simulink model "turbo_controller"  (R2025a)
settings: Solver=FixedStepAuto  StartTime=0.0  StopTime=inf  FixedStep=0.001  RelTol=1e-3
PostLoadFcn:
  | % 自动定位同目录CubeMX文件；不需要外部初始化脚本。
  | codertarget.data.setParameterValue('turbo_controller','STM32CubeMX.ProjectFile',fullfile(fileparts(get_param('turbo_controller','FileName')),'turbo_f407.ioc'));
InitFcn:
  | % 中文说明：按原控制器字段与类型创建三组接口总线；控制参数已内嵌。
  | tc_names=["EValve_Cycle" "EValve_Open" "Eblast_Cycle" "Eblast_Open" "Motor_Cycle" "Motor_Open" "EValve_Enable" "Eblast_Enable" "Motor_Enable" "SWO_Firework" "SWO_BleedAir" "EngineState" "Flag_ECUReset_Clear" "Flag_ECUReset_Save" "Flag_Reset_Enable" "Accelerator" "Nc_dem" "Nc"]; tc_types=["uint16" "uint16" "uint16" "uint16" "uint16" "uint16" "uint8" "uint8" "uint8" "uint8" "uint8" "uint8" "uint8" "uint8" "uint8" "single" "single" "single"];
  | for tc_k=1:numel(tc_names)
  |  tc_e(tc_k)=Simulink.BusElement; tc_e(tc_k).Name=char(tc_names(tc_k)); tc_e(tc_k).DataType=char(tc_types(tc_k));
  | end
  | EngineControl_Out=Simulink.Bus; EngineControl_Out.DataScope='Exported'; EngineControl_Out.Elements=tc_e;
  | clear tc_e tc_names tc_types tc_k
  | tc_names=["savedata1" "savedata2" "savedata3" "savedata4" "savedata5" "savedata6" "savedata7" "savedata8" "savedata9" "savedata10" "savedata11" "savedata12" "savedata13" "savedata14" "savedata15" "savedata16" "savedata17" "savedata18" "savedata19" "savedata20" "savedata21" "savedata22" "savedata23" "savedata24" "savedata25"]; tc_types=["single" "single" "single" "single" "single" "single" "single" "single" "single" "single" "single" "single" "single" "single" "single" "single" "single" "single" "single" "single" "single" "single" "single" "single" "single"];
  | for tc_k=1:numel(tc_names)
  |  tc_e(tc_k)=Simulink.BusElement; tc_e(tc_k).Name=char(tc_names(tc_k)); tc_e(tc_k).DataType=char(tc_types(tc_k));
  | end
  | SaveData_Out=Simulink.Bus; SaveData_Out.DataScope='Exported'; SaveData_Out.Elements=tc_e;
  | clear tc_e tc_names tc_types tc_k
  | tc_names=["senddata1" "senddata2" "senddata3" "senddata4" "senddata5" "senddata6" "senddata7" "senddata8" "senddata9" "senddata10" "senddata11" "senddata12" "senddata13" "senddata14" "senddata15" "senddata16" "senddata17" "senddata18" "senddata19" "senddata20" "senddata21" "senddata22" "senddata23" "senddata24" "senddata25" "senddata26" "senddata27" "senddata28" "senddata29"]; tc_types=["uint8" "uint8" "uint8" "uint8" "uint8" "uint8" "uint8" "uint8" "uint8" "uint8" "uint8" "uint8" "uint8" "uint8" "uint8" "uint8" "uint8" "uint8" "uint8" "uint8" "uint8" "uint8" "uint8" "uint8" "uint8" "uint8" "uint8" "uint8" "uint8"];
  | for tc_k=1:numel(tc_names)
  |  tc_e(tc_k)=Simulink.BusElement; tc_e(tc_k).Name=char(tc_names(tc_k)); tc_e(tc_k).DataType=char(tc_types(tc_k));
  | end
  | SendData_Out=Simulink.Bus; SendData_Out.DataScope='Exported'; SendData_Out.Elements=tc_e;
  | clear tc_e tc_names tc_types tc_k
  | 
  | % 以下为接口中文说明；只设置描述，不改变数值或数据类型。
  | EngineControl_Out.Description='执行控制输出（阀、电机、点火、状态及复位请求）';
  | tc_cn=["EValve_Cycle（主油阀周期计数（每计数2毫秒））" "EValve_Open（主油阀开通计数（每计数2毫秒））" "Eblast_Cycle（副油阀周期计数（每计数2毫秒））" "Eblast_Open（副油阀开通计数（每计数2毫秒））" "Motor_Cycle（起动电机周期计数）" "Motor_Open（起动电机开通计数）" "EValve_Enable（主油阀驱动使能）" "Eblast_Enable（副油阀驱动使能）" "Motor_Enable（起动电机使能）" "SWO_Firework（点火器使能（1开））" "SWO_BleedAir（引气阀使能（1开））" "EngineState（发动机状态）" "Flag_ECUReset_Clear（清除复位恢复状态请求）" "Flag_ECUReset_Save（保存复位恢复数据请求）" "Flag_Reset_Enable（处理器软件复位请求）" "Accelerator（油门／油泵给定控制量）" "Nc_dem（控制目标转速）" "Nc（发动机反馈转速（转每分））"];
  | tc_elements=EngineControl_Out.Elements;
  | for tc_k=1:numel(tc_cn)
  |  tc_elements(tc_k).Description=char(tc_cn(tc_k));
  | end
  | EngineControl_Out.Elements=tc_elements;
  | clear tc_cn tc_elements tc_k
  | SaveData_Out.Description='25项运行记录；字段含义按当前模型数据来源解释';
  | tc_cn=["savedata1（指令回显记录）" "savedata2（入口总温记录（℃））" "savedata3（电源电压记录）" "savedata4（排气温度记录（℃））" "savedata5（标定燃油压力记录）" "savedata6（副油阀占空比记录（％））" "savedata7（主油阀占空比记录（％））" "savedata8（温度修正转速记录）" "savedata9（开关输出及反馈位域）" "savedata10（物理转速记录）" "savedata11（油泵目标给定原始值）" "savedata12（起动电机占空比记录（％））" "savedata13（发动机状态码记录）" "savedata14（故障告警位域记录）" "savedata15（模型记录帧序号）" "savedata16（处理器温度记录（℃））" "savedata17（装订转速记录（沿用旧电源字段名））" "savedata18（导航高度记录）" "savedata19（飞行空速记录）" "savedata20（主阀旧记录位（恒零保留））" "savedata21（第21项保留记录（恒零））" "savedata22（保留记录项22）" "savedata23（保留记录项23）" "savedata24（保留记录项24）" "savedata25（保留记录项25）"];
  | tc_elements=SaveData_Out.Elements;
  | for tc_k=1:numel(tc_cn)
  |  tc_elements(tc_k).Description=char(tc_cn(tc_k));
  | end
  | SaveData_Out.Elements=tc_elements;
  | clear tc_cn tc_elements tc_k
  | SendData_Out.Description='29字段回传及外设命令接口；板端上位机帧只取第3至27字段';
  | tc_cn=["senddata1（回传发送允许标志（不直接上线路））" "senddata2（回传载荷长度25字节）" "senddata3（回传指令回显字节）" "senddata4（总温编码字节（℃＋80））" "senddata5（电源电压编码字节）" "senddata6（排温编码高字节）" "senddata7（排温编码低字节）" "senddata8（燃油压力编码高字节）" "senddata9（燃油压力编码低字节）" "senddata10（副油阀占空比字节（％））" "senddata11（主油阀占空比字节（％））" "senddata12（修正转速编码高字节）" "senddata13（修正转速编码低字节）" "senddata14（驱动及反馈状态位域）" "senddata15（物理转速编码高字节）" "senddata16（物理转速编码低字节）" "senddata17（油泵目标给定高字节（串口二使用））" "senddata18（油泵目标给定低字节（串口二使用））" "senddata19（起动电机占空比命令（串口一使用））" "senddata20（发动机状态码字节）" "senddata21（故障告警位域字节）" "senddata22（帧序号占位（板端另行填写））" "senddata23（处理器温度编码（℃＋50））" "senddata24（控制目标转速编码高字节）" "senddata25（控制目标转速编码低字节）" "senddata26（占位字节（板端改填实测泵速高字节））" "senddata27（占位字节（板端改填实测泵速低字节））" "senddata28（装订转速高字节（本板未发送））" "senddata29（装订转速低字节（本板未发送））"];
  | tc_elements=SendData_Out.Elements;
  | for tc_k=1:numel(tc_cn)
  |  tc_elements(tc_k).Description=char(tc_cn(tc_k));
  | end
  | SendData_Out.Elements=tc_elements;
  | clear tc_cn tc_elements tc_k
  | 
  | 
  | % FRAM模块化事务：接口类型和上电初始状态，随模型保存，无外部初始化文件。
  | clear FM_elements
  | FM_elements(1)=Simulink.BusElement;FM_elements(1).Name='phase';FM_elements(1).DataType='uint8';FM_elements(1).Dimensions=[1 1];FM_elements(1).Description='phase（当前事务阶段）';
  | FM_elements(2)=Simulink.BusElement;FM_elements(2).Name='a';FM_elements(2).DataType='uint8';FM_elements(2).Dimensions=[64 1];FM_elements(2).Description='a（启动时缓存的首区64字节）';
  | FM_elements(3)=Simulink.BusElement;FM_elements(3).Name='active';FM_elements(3).DataType='uint16';FM_elements(3).Dimensions=[1 1];FM_elements(3).Description='active（当前有效记录区地址）';
  | FM_elements(4)=Simulink.BusElement;FM_elements(4).Name='generation';FM_elements(4).DataType='uint32';FM_elements(4).Dimensions=[1 1];FM_elements(4).Description='generation（当前有效记录代号）';
  | FM_elements(5)=Simulink.BusElement;FM_elements(5).Name='record';FM_elements(5).DataType='uint8';FM_elements(5).Dimensions=[64 1];FM_elements(5).Description='record（本次冻结的待写记录）';
  | FM_elements(6)=Simulink.BusElement;FM_elements(6).Name='addr';FM_elements(6).DataType='uint16';FM_elements(6).Dimensions=[1 1];FM_elements(6).Description='addr（本次备用写入地址）';
  | FM_elements(7)=Simulink.BusElement;FM_elements(7).Name='lastSave';FM_elements(7).DataType='single';FM_elements(7).Dimensions=[1 1];FM_elements(7).Description='lastSave（上次开始保存的秒数）';
  | FM_elements(8)=Simulink.BusElement;FM_elements(8).Name='lastState';FM_elements(8).DataType='uint8';FM_elements(8).Dimensions=[1 1];FM_elements(8).Description='lastState（上次保存时的发动机状态）';
  | FM_elements(9)=Simulink.BusElement;FM_elements(9).Name='boot';FM_elements(9).DataType='boolean';FM_elements(9).Dimensions=[1 1];FM_elements(9).Description='boot（启动记录是否允许恢复）';
  | FM_elements(10)=Simulink.BusElement;FM_elements(10).Name='consumed';FM_elements(10).DataType='boolean';FM_elements(10).Dimensions=[1 1];FM_elements(10).Description='consumed（本次启动恢复通知是否已发送）';
  | FM_elements(11)=Simulink.BusElement;FM_elements(11).Name='payload';FM_elements(11).DataType='uint8';FM_elements(11).Dimensions=[20 1];FM_elements(11).Description='payload（当前20字节恢复内容）';
  | ... (+35 lines)
model workspace (MAT data in the model file):
  CRC16_Table_Reference = [0 4129 8258 12387 16516 20645 24774 28903 33032 37161 41290 45419 ... (256 elements, 256x1)]
  PE_Kaer = [0.15402 0.15402 0.12264 0.10076 0.09481 0.07601 0.07111 0.0569 0.05198 0.04926 0.05308 0.04325 ... (13 elements, 1x13)]
  PE_Nr = [21.2982 61.4260372 67.7475458 72.7394382 76.845934 80.6988798 83.8449282 86.6491912 88.9382406 89.178606 91.1938214 93.4068058 ... (13 elements, 1x13)]
  PE_Pump_Translate = 33.5999984741
  PE_RotaSpeed_Translate = 860
  PE_Taer = [0.4939154 0.4939154 0.40780982 0.34066978 0.31622756 0.30405716 0.34300244 0.26785022 0.37393554 0.23914836 0.44563948 0.31044662 ... (13 elements, 1x13)]
  PF_ACCFULLRANGE = 3360
  PF_Flag_ECUReset = 0
  PF_Flag_rx_suc = 1
  PF_Gear_Info = [40000; 45000; 50000; 55000; 57000; 59000; 60000; 61000; 61000; 61000; 61000; 61000]
  PF_K_TiaoJie = 1
  PF_Kpu = 10
  PF_MySet_Rxdata = [0 0 0 0 0 0 0 0 0 0 0 0 ... (50 elements, 50x1)]
  PF_MyUsart1_Rxdata = [0 0 0 0 0 0 0 0 0 0 0 0 ... (50 elements, 50x1)]
  PF_MyUsart2_Rxdata = [0 0 0 0 0 0 0 0 0 0 0 0 ... (50 elements, 50x1)]
  PF_Reset_Information = [0 0 0 0 0 0 0 0 0 0 0 0 ... (20 elements, 20x1)]
  PF_Sensor_X1_T4 = [0 4095]
  PF_Sensor_X2_T4 = [0 1.66666698456]
  PF_Sensor_X3_T4 = [0 504 999 1497 2010 2529 3051 3568 4076 4571 4959]
  PF_Sensor_X_P2 = [0.5 3]
  PF_Sensor_X_Poil = [0.5 3]
  PF_Sensor_X_T1t = [-50 300]
  PF_Sensor_X_Vpower = [0 3]
  PF_Sensor_X_Vpump = [0 3]
  PF_Sensor_Y1_T4 = [0 3]
  PF_Sensor_Y2_T4 = [0 5000]
  PF_Sensor_Y3_T4 = [0 100 200 300 400 500 600 700 800 900 980]
  PF_Sensor_Y_P2 = [0 1000]
  PF_Sensor_Y_Poil = [0 1000]
  PF_Sensor_Y_T1t = [-50 300]
  PF_Sensor_Y_Vpower = [0 33]
  PF_Sensor_Y_Vpump = [0 33]
  PG_CtrlMode_CloseLoop : mpt.Parameter (value not decoded)
  PG_CtrlMode_ManualAcc : mpt.Parameter (value not decoded)
  PG_CtrlMode_Origin : mpt.Parameter (value not decoded)
  PG_CtrlMode_Start : mpt.Parameter (value not decoded)
  PG_CtrlMode_Stop : mpt.Parameter (value not decoded)
  PG_ES_Clp : mpt.Parameter (value not decoded)
  PG_ES_EngStart : mpt.Parameter (value not decoded)
  PG_ES_Manual : mpt.Parameter (value not decoded)
  PG_ES_Origin : mpt.Parameter (value not decoded)
  PG_ES_Stop : mpt.Parameter (value not decoded)
  PG_Instr_BleedAirSet : mpt.Parameter (value not decoded)
  PG_Instr_CloseLoop : mpt.Parameter (value not decoded)
  PG_Instr_ECUReSet : mpt.Parameter (value not decoded)
  PG_Instr_EValveSet : mpt.Parameter (value not decoded)
  PG_Instr_EblastSet : mpt.Parameter (value not decoded)
  PG_Instr_Erase : mpt.Parameter (value not decoded)
  PG_Instr_FireWorkSet : mpt.Parameter (value not decoded)
  PG_Instr_ManualPlus : mpt.Parameter (value not decoded)
  PG_Instr_ManualrReduce : mpt.Parameter (value not decoded)
  PG_Instr_MotorSet : mpt.Parameter (value not decoded)
  PG_Instr_OilSet : mpt.Parameter (value not decoded)
  PG_Instr_SelfCheck : mpt.Parameter (value not decoded)
  PG_Instr_Start : mpt.Parameter (value not decoded)
  PG_Instr_Stop : mpt.Parameter (value not decoded)
  PG_Instr_StopZero : Simulink.Parameter (value not decoded)
  PG_Location_Air : Simulink.Parameter (value not decoded)
  PG_Location_Gnd : Simulink.Parameter (value not decoded)
  PG_ServoCtrlMode_CloseLoop : Simulink.Parameter (value not decoded)
  PG_ServoCtrlMode_CloseLoopMax : Simulink.Parameter (value not decoded)
  PG_ServoCtrlMode_CloseLoopMin : Simulink.Parameter (value not decoded)
  PG_ServoCtrlMode_ManualAcc : Simulink.Parameter (value not decoded)
  PG_ServoCtrlMode_ManualAccMax : Simulink.Parameter (value not decoded)
  PG_ServoCtrlMode_ManualAccMin : Simulink.Parameter (value not decoded)
  PG_SpeedDot_Permit : Simulink.Parameter (value not decoded)
  PL_EngineModel_Actuator = [0 10 100]
  PL_EngineModel_EngineStar_Press_P2 = [1013 1098.4 1099.144828 1099.931034 1103.613793 1162.662069 1143.793103 1131.006897 1123.186207 1117.6 1114 1111.806897 ... (127 elements, 1x127)]
  PL_EngineModel_EngineStar_RotaSpeed = [200 2000 9584 9660 10220 10240 10260 10288 10308 10368 10380 10408 ... (127 elements, 1x127)]
  PL_EngineModel_EngineStar_Temp_Exhaust = [128 129 129.1 130 131 131.1 132 133 134 134.1 135 135.1 ... (127 elements, 1x127)]
  PL_EngineModel_EngineStar_Time = [0.05 0.1 0.15 0.2 0.25 0.3 0.35 0.4 0.45 0.5 0.55 0.6 ... (127 elements, 1x127)]
  PL_EngineModel_IdleAbove_Nr = [0 21.2982 61.4260372 67.7475458 72.7394382 76.845934 80.6988798 83.8449282 86.6491912 88.9382406 89.178606 91.1938214 ... (14 elements, 1x14)]
  PL_EngineModel_IdleAbove_P2r = [0.986923266716 1.57907722675 1.81593881076 1.99358499877 2.23044658278 2.43770046879 2.65482358747 2.84233900814 3.03972366149 3.18776215149 3.25684678016 3.3950160375 ... (14 elements, 1x14)]
  PL_EngineModel_IdleAbove_Tempr = [0.0536001429337 1.07200285867 1.63301768805 1.63659103091 1.66875111667 1.72592460247 1.77595140254 1.86171163123 1.95461854565 2.03323208862 2.03323208862 2.13685903162 ... (14 elements, 1x14)]
  PL_EngineModel_IdleAbove_Ter = [0.42434128 0.42434128 0.42434128 0.30669408 0.23570008 0.22150128 0.1997974 0.23803274 0.16115638 0.24279948 0.13600422 0.31308354 ... (14 elements, 1x14)]
  PL_EngineModel_IdleAbove_Wfr = [0 10.142 23.8337 27.8905 31.9473 36.0041 40.0609 44.1177 48.1745 52.2313 52.7384 56.7952 ... (14 elements, 1x14)]
  PL_EngineModel_Press_P2 = [400 400 400 400 400 400 400 400 400 400]
  PL_EngineModel_Rotaspeed = [0 20000 96400]
  PL_EngineModel_Temp_Exhaust = [500 500 500 500 500 500 500 500 500 500]
  PL_Kaer = [0.1 0.1 0.1 0.1 0.1 0.1]
  PL_Nr = [50 60 70 80 90 100]
  PL_Taer = [0.1 0.1 0.1 0.1 0.1 0.1]
  Sig : Simulink.Signal (value not decoded)
  Ts_ms : Simulink.Parameter (value not decoded)
  false : Simulink.Parameter (value not decoded)
  true : Simulink.Parameter (value not decoded)
symbols that are objects in the model workspace (value not decoded): PG_CtrlMode_CloseLoop, PG_CtrlMode_ManualAcc, PG_CtrlMode_Origin, PG_CtrlMode_Start, PG_CtrlMode_Stop, PG_ES_Clp, PG_ES_EngStart, PG_ES_Manual, PG_ES_Origin, PG_ES_Stop, PG_Instr_BleedAirSet, PG_Instr_CloseLoop, PG_Instr_EblastSet, PG_Instr_ECUReSet, PG_Instr_Erase, PG_Instr_EValveSet, PG_Instr_FireWorkSet, PG_Instr_ManualPlus, PG_Instr_ManualrReduce, PG_Instr_MotorSet, PG_Instr_OilSet, PG_Instr_SelfCheck, PG_Instr_Start, PG_Instr_Stop, PG_Instr_StopZero, PG_ServoCtrlMode_CloseLoop, PG_ServoCtrlMode_CloseLoopMax, PG_ServoCtrlMode_CloseLoopMin, PG_ServoCtrlMode_ManualAcc, PG_ServoCtrlMode_ManualAccMax, PG_ServoCtrlMode_ManualAccMin, Ts_ms
libraries: simulink x97, stm32blockslib x10, stm32f4xxblockslib x8
(part 11 of 26)

== system turbo_controller/BoardInput_输入换算与协议解析/In04_Capture（捕获间隔缓存）/Step03_计算间隔并更新环形缓存 ==
  note: 对一项捕获完成回卷差分和缓存更新
      |
      | 输入为上一捕获、旧十项缓存、旧写入位置、旧有效数、旧最近时间，以及本次Capture、Seconds和Ac
      | tive。
      |
      | 六步各做一件事：算回卷后的间隔、判断能否接受、生成缓存候选值、计算下一写入位置、计算有效数
      | 量、最后按许可提交状态。
      |
      | 关键规则有两条：只要Active为真就更新Previous；但只有Active为真且间隔>0，才更新Ring、Index
      | 、Count和LastTime。重复读数的零间隔不会增加记录，也不刷新最近有效时间。
      |
      | 例：上次65530、这次4，间隔为10；若本项有效，就存10并更新状态。若本项无效，即使算出了10，也
      | 保留全部旧状态。输出回到In04的历史记忆供下一项使用，不是给硬件发送命令。
  Previous（上次捕获计数）_374 : Inport  OutDataTypeStr=uint32
  Ring（十项间隔缓存）_375 : Inport  Port=2  OutDataTypeStr=single
  Index（下一写入位置）_376 : Inport  Port=3  OutDataTypeStr=uint8
  Count（有效间隔个数）_377 : Inport  Port=4  OutDataTypeStr=uint8
  LastTime（最近有效脉冲时间）_378 : Inport  Port=5  OutDataTypeStr=single
  Capture（当前捕获计数）_379 : Inport  Port=6  OutDataTypeStr=uint16
  Seconds（当前秒数）_380 : Inport  Port=7  OutDataTypeStr=double
  Active（本项捕获有效）_381 : Inport  Port=8  OutDataTypeStr=boolean
  Step01_计算回卷后的脉冲间隔 : Subsystem  Description=|
      | 第一步：把16位捕获读数换成正向间隔
      | 
      | 先转换当前与上次读数的类型，避免直接用无符号数相减造成负差丢失。再计算：
      | 间隔=mod(本次Capture-上次Previous,65536)。
      | 
      | 当前配置每个计数为1微秒。例：上次1000、当前2000，得到1000微秒；上次65530、当前4，得到10微秒。65536来自16位计数器的一个完整回卷周期。
      | 
      | 本步骤只产生候选间隔，不检查Active，也不写缓存。回卷差分只保留模65536的结果，并没有额外累计跨越多个完整回卷的时间。
      | 
      | 初始Previous沿用原模型的0，所以第一条正读数会相对0求差；本次拆分没有新增“第一脉冲只初始化”的规则。
  Step02_判断间隔是否有效 : Subsystem  Description=|
      | 第二步：决定这个间隔能否新增一条记录
      | 
      | 允许保存=Active AND 间隔>0。
      | 
      | Active说明本项确实属于本批新捕获，间隔>0排除重复读数。例：本次捕获和上次相同，间隔0，虽然Active为真，也不新增间隔、不推进环形位置、不增加数量、不刷新最近有效时间。
      | 
      | 没有有效新项时，即使候选差分非0，也不采用。这个许可送最后的提交步骤；本步骤自身没有记忆，也不判断转速是否超限。
  Step03_生成缓存写入候选值 : Subsystem  Description=|
      | 第三步：准备一份只改一项的缓存候选值
      | 
      | 按当前Index，把本次间隔写进旧Ring对应的位置，其余九项保留。Index是1～10的环形写入位置，不是本批捕获数组的序号。
      | 
      | 例：Index=4、间隔1000，则候选数组只把第4项换成1000。即使第二步不允许保存，这里也可算出候选数组；最终会由第六步选择旧缓存，候选值不会生效。
      | 
      | 这里的Assignment不增加数组长度，不求平均，也不清空其他项。
  Step04_计算下次环形写入位置 : Subsystem  Description=|
      | 第四步：准备下一次应覆盖的环形位置
      | 
      | 候选下一位置=mod(本次Index,10)+1。
      | 
      | Index=1得到2，Index=9得到10，Index=10得到1。这样十项写满后继续从第1项覆盖最旧记录。
      | 
      | 本步骤只算候选位置；只有第六步收到保存许可才采用它。零间隔或无效捕获不会因为这里已经算出下一位置就推进缓存。
  Step05_计算已保存间隔数量 : Subsystem  Description=|
      | 第五步：准备累计有效间隔数量
      | 
      | 候选数量=min(旧Count+1,10)。
      | 
      | 未填满时，每接受一个正间隔增加1；达到10后保持10。例：旧数量8得到候选9，旧数量10仍得到10。数量到10不会让后续数据停止写入，环形位置仍继续轮转覆盖。
      | 
      | 本步骤不是统计本批有几个捕获。它计算缓存有效条数的候选值，只有第六步有保存许可才提交；否则继续旧Count。
  Step06_有效才提交并更新时间 : Subsystem  Description=|
      | 第六步：按许可提交候选状态，并记录新鲜程度
      | 
      | 分别选择两类状态：
      | Previous：Active为真就采用当前Capture，否则保持旧Previous。
      | Ring、Index、Count、LastTime：只有第二步允许保存时，才采用第三～五步候选值，并把LastTime更新为当前Seconds；否则全部保持旧值。
      | 
      | 例：有效捕获但与上次相同，Previous仍更新到当前读数，其他四项不变。这种情况下不会伪造一条0间隔，也不会让后面的超时判断误以为又收到了一条有效间隔。
      | 
      | LastTime记录的是本批处理时刻，单位秒；同一批多个捕获共用这一时刻。它不等同于每个脉冲精确的硬件到达时刻，精确间隔来自计数差分。
      | 
      | 五项输出交外层记忆。本处没有新增延迟，没有直接输出转速，也不负责选择电机反馈或捕获测速。
  Previous（下次差分基准）_405 : Outport
  Ring（更新后的间隔缓存）_407 : Outport  Port=2
  Index（下次写入位置）_409 : Outport  Port=3
  Count（更新后的有效个数）_411 : Outport  Port=4
  LastTime（最近有效脉冲时间）_414 : Outport  Port=5
  wires:
  Step06_有效才提交并更新时间/1(输出1_下一差分基准) -> Previous（下次差分基准）_405/1
  Ring（十项间隔缓存）_375/1 -> Step03_生成缓存写入候选值/2(输入2_旧十项间隔缓存), Step06_有效才提交并更新时间/7(输入7_旧十项间隔缓存)  "旧十项间隔缓存"
  Capture（当前捕获计数）_379/1 -> Step06_有效才提交并更新时间/1(输入1_本项捕获读数), Step01_计算回卷后的脉冲间隔/1(输入1_本项捕获读数)  "本项捕获读数"
  Previous（上次捕获计数）_374/1 -> Step06_有效才提交并更新时间/4(输入4_上一捕获读数), Step01_计算回卷后的脉冲间隔/2(输入2_上一捕获读数)  "上一捕获读数"
  Step01_计算回卷后的脉冲间隔/1(输出1_回卷后的脉冲间隔) -> Step02_判断间隔是否有效/1(输入1_回卷后的脉冲间隔), Step03_生成缓存写入候选值/1(输入1_回卷后的脉冲间隔)  "回卷后的脉冲间隔"
  Count（有效间隔个数）_377/1 -> Step06_有效才提交并更新时间/11(输入11_累计有效间隔数), Step05_计算已保存间隔数量/1(输入1_累计有效间隔数)  "累计有效间隔数"
  Active（本项捕获有效）_381/1 -> Step06_有效才提交并更新时间/3(输入3_本项捕获有效), Step02_判断间隔是否有效/2(输入2_本项捕获有效)  "本项捕获有效"
  Seconds（当前秒数）_380/1 -> Step06_有效才提交并更新时间/2(输入2_当前处理时刻_秒)  "当前处理时刻_秒"
  Index（下一写入位置）_376/1 -> Step06_有效才提交并更新时间/9(输入9_当前环形写入位置), Step04_计算下次环形写入位置/1(输入1_当前环形写入位置), Step03_生成缓存写入候选值/3(输入3_当前环形写入位置)  "当前环形写入位置"
  Step02_判断间隔是否有效/1(输出1_允许保存正间隔) -> Step06_有效才提交并更新时间/6(输入6_允许保存正间隔)  "允许保存正间隔"
  Step06_有效才提交并更新时间/3(输出3_下一环形写入位置) -> Index（下次写入位置）_409/1
  Step03_生成缓存写入候选值/1(输出1_候选十项间隔缓存) -> Step06_有效才提交并更新时间/5(输入5_候选十项间隔缓存)  "候选十项间隔缓存"
  Step04_计算下次环形写入位置/1(输出1_候选下次写入位置) -> Step06_有效才提交并更新时间/8(输入8_候选下次写入位置)  "候选下次写入位置"
  Step05_计算已保存间隔数量/1(输出1_候选有效间隔数量) -> Step06_有效才提交并更新时间/10(输入10_候选有效间隔数量)  "候选有效间隔数量"
  LastTime（最近有效脉冲时间）_378/1 -> Step06_有效才提交并更新时间/12(输入12_上次有效间隔时刻)  "上次有效间隔时刻"
  Step06_有效才提交并更新时间/2(输出2_更新后的十项间隔) -> Ring（更新后的间隔缓存）_407/1
  Step06_有效才提交并更新时间/4(输出4_更新后的有效间隔数) -> Count（更新后的有效个数）_411/1
  Step06_有效才提交并更新时间/5(输出5_最近有效间隔处理时刻) -> LastTime（最近有效脉冲时间）_414/1

== system turbo_controller/BoardInput_输入换算与协议解析/In04_Capture（捕获间隔缓存）/Step04_整理间隔数量和时间输出 ==
  note: 第四步：整理三个对外输出的形状，不再次计算
      |
      | 将Step03输出的十项Ring整理为原工程的一维向量接口；累计有效数量和最近有效时间按原来要求整理
      | 为标量形状。
      |
      | 数值不变、单位不变，也不做新的滤波。Periods仍是计数间隔，当前配置下可按微秒解释；Count仍为
      | 0～10；LastTime仍为秒。
      |
      | 例如Ring中一项1000经过此处还是1000，不会变成1000转/分。真正的转速换算在后面的CaptureSpeed
      | ，超时判断在Status；本块只保证连接双方看到的数组形状与修改前一致。
  输入1_更新后的有效间隔数 : Inport
  输入2_最近有效间隔处理时刻 : Inport  Port=2
  输入3_更新后的十项间隔 : Inport  Port=3
  Format（保持原输出维度）_2 : Reshape
  Format（保持原输出维度）_3 : Reshape
  Vector1D（保持原一维向量接口）_1 : Reshape
  输出1_Vector1D（保持原一维向量接口） : Outport
  输出2_Format（保持原输出维度） : Outport  Port=2
  输出3_Format（保持原输出维度） : Outport  Port=3
  wires:
  Format（保持原输出维度）_3/1 -> 输出3_Format（保持原输出维度）/1
  Format（保持原输出维度）_2/1 -> 输出2_Format（保持原输出维度）/1
  Vector1D（保持原一维向量接口）_1/1 -> 输出1_Vector1D（保持原一维向量接口）/1
  输入3_更新后的十项间隔/1 -> Vector1D（保持原一维向量接口）_1/1
  输入2_最近有效间隔处理时刻/1 -> Format（保持原输出维度）_3/1
  输入1_更新后的有效间隔数/1 -> Format（保持原输出维度）_2/1

== system turbo_controller/BoardInput_输入换算与协议解析/In05_Speed（转速来源选择与滤波）/CaptureSpeed（去极值估算转速）_19 ==
  note: 把最近脉冲间隔换算成转速：先筛数据，再去极值，最后计算
      |
      | 输入Periods最多十项，Count=n说明前几项有效。四步分别是：排除空位、去掉一个最大值和一个最小
      | 值、检查分母并避免除零、按每转3脉冲换算RPM。
      |
      | 去极值后的和S=有效间隔之和-最大有效间隔-最小有效间隔。
      | 转速=60000000×(n-2)/(3×S)，间隔采用微秒时，输出单位为转/分。
      |
      | 例如十项都为1000微秒，去掉两项后S=8000，转速=60000000×8/(3×8000)=20000。去极值减轻单个偏大
      | /偏小间隔的影响，不是无条件识别所有错误脉冲。
      |
      | 本模块Valid只表示S>0。至少有3项的要求、最近脉冲是否超时、是否优先采用电机串口反馈，由外层S
      | tatus和Select决定。数据不足时即使这里有一个数，也不能绕过这些条件直接用作控制反馈。
  Periods（最近十项间隔）_444 : Inport  OutDataTypeStr=single
  Count（有效项数）_445 : Inport  Port=2  OutDataTypeStr=uint8
  Step01_选出有效间隔 : Subsystem  Description=|
      | 第一步：标出前n个有效位置，求和时把其他位置变0
      | 
      | 缓存固定十项，但刚开始未必填满。将序号1～10分别与Count比较，序号≤Count才标记为有效。
      | 
      | 求和用的数组：有效位置保留原间隔，无效位置填0。与此同时把有效位置掩码送下一步，用于寻找真正有效项中的最大值和最小值。
      | 
      | 例：Count=3，缓存[1000,1100,900,0,…]，求和数组只采用前三项，后七项不作为测量。Count是间隔条数，不是时间，也不是每转脉冲数。
      | 
      | 本步骤不改写原缓存，只生成本次计算用的数据与掩码。
  Step02_去掉最大最小再求和 : Subsystem  Description=|
      | 第二步：去掉一个最大间隔和一个最小间隔
      | 
      | 先对第一步的求和数组求总和。找最大值时，无效位置用0占位；找最小值时，无效位置用single最大有限值占位，避免未填满缓存的0被误当作最小有效间隔。
      | 
      | S=有效间隔总和-最大有效间隔-最小有效间隔。
      | 例：[900,1000,1100]的总和3000，去掉1100和900，S=1000；剩下一项用于估速。若十项都是1000，去掉其中两项，S=8000。
      | 
      | 每种极值只减一项；即使有多个相同最大值，也不是全部删除。这里求的是剩余间隔总和，还没有除以n-2；第四步会把剩余项数并入转速公式。
  Step03_检查分母并防止除零 : Subsystem  Description=|
      | 第三步：判断去极值后的总和能否作分母
      | 
      | Valid=(S>0)。有效时把S交给下一步；无效时，内部改用1作为安全分母，避免除零。
      | 
      | 安全分母1只是防止算术错误，不能表示测量间隔为1微秒。Valid为假时，后面的数值输出不可单独当作有效转速。
      | 
      | 本步骤也不判断Count≥3。这个数量条件在外层Status；只有数量、分母和时间条件都满足，外层才会采用捕获估速。
  Step04_按每转三脉冲计算转速 : Subsystem  Description=|
      | 第四步：将剩余间隔总和换算成每分钟转数
      | 
      | 输入有效间隔数n与前一步给出的安全分母S。先求剩余条数n-2，再计算：
      | 转速=60000000×(n-2)/(3×S)。
      | 
      | 60000000是一分钟的微秒数；3表示本工程每转3个脉冲；S/(n-2)相当于去极值后的平均脉冲间隔。这里没有另外的隐含乘100或除100。
      | 
      | 例：n=10、S=8000微秒，得到20000转/分。这个数是捕获候选转速，最终仍由外层的数量判断、超时判断和来源选择决定是否使用。不能因为采用了安全分母就忽略Valid。
  Speed（定时器估算转速）_471 : Outport
  Valid（估算分母有效）_472 : Outport  Port=2
  wires:
  Step03_检查分母并防止除零/2(输出2_分母为正) -> Valid（估算分母有效）_472/1
  Step04_按每转三脉冲计算转速/1(输出1_捕获候选转速_RPM) -> Speed（定时器估算转速）_471/1
  Step03_检查分母并防止除零/1(输出1_用于计算的安全分母) -> Step04_按每转三脉冲计算转速/2(输入2_用于计算的安全分母)  "用于计算的安全分母"
  Step02_去掉最大最小再求和/1(输出1_去极值后间隔总和) -> Step03_检查分母并防止除零/1(输入1_去极值后间隔总和)  "去极值后间隔总和"
  Step01_选出有效间隔/2(输出2_无效项已清零的求和数据) -> Step02_去掉最大最小再求和/3(输入3_无效项已清零的求和数据)  "无效项已清零的求和数据"
  Step01_选出有效间隔/1(输出1_有效位置掩码) -> Step02_去掉最大最小再求和/2(输入2_有效位置掩码)  "有效位置掩码"
  Periods（最近十项间隔）_444/1 -> Step02_去掉最大最小再求和/1(输入1_原十项间隔缓存), Step01_选出有效间隔/2(输入2_原十项间隔缓存)  "原十项间隔缓存"
  Count（有效项数）_445/1 -> Step01_选出有效间隔/1(输入1_有效间隔条数), Step04_按每转三脉冲计算转速/1(输入1_有效间隔条数)  "有效间隔条数"

== system turbo_controller/BoardInput_输入换算与协议解析/In05_Speed（转速来源选择与滤波）/Clock20ms（二十毫秒更新节拍）_18 ==
  note: 从秒数产生每二十毫秒一次的许可
      |
      | 本模块收到当前模型时间Seconds。先乘1000换成毫秒，再对20取余，判断余数是否小于1：
      | 工作许可 = mod(Seconds×1000,20)<1。
      |
      | 在父级1 ms离散调用下，约在0、20、40、60 ms等时刻为真，中间毫秒为假。用“小于1”表示当前1 m
      | s时间格，避免把它理解成连续时间的一次精确相等判断。
      |
      | 这只是一个布尔许可，不会让模型等待或暂停。转速选择用它决定何时更新Speed，回传组帧用它决定
      | 何时生成新帧；其他1 ms任务继续正常运行。
  Seconds（当前秒数）_9 : Inport  OutDataTypeStr=double
  Constant（常量）_10 : Constant  Value=1000  OutDataTypeStr=double
  Constant（常量）_13 : Constant  Value=20  OutDataTypeStr=double
  Constant（常量）_15 : Constant  Value=0  OutDataTypeStr=double
  Every20ms（20毫秒更新许可）_16 : RelationalOperator  Operator===  OutDataTypeStr=boolean  RndMeth=Simplest  InputSameDT=off
  Milliseconds（秒换算为毫秒）_11 : Product  Inputs=**  SaturateOnIntegerOverflow=on  OutDataTypeStr=Inherit: Same as first input
  Phase20（20毫秒相位）_14 : Math  Operator=mod
  RoundTime（按原规则取整）_12 : Rounding  Operator=round
  Every20ms（二十毫秒更新许可）_17 : Outport
  wires:
  Seconds（当前秒数）_9/1 -> Milliseconds（秒换算为毫秒）_11/1  "Seconds（当前秒数）"
  Every20ms（20毫秒更新许可）_16/1 -> Every20ms（二十毫秒更新许可）_17/1  "Every20ms（20毫秒更新许可）"
  Constant（常量）_10/1 -> Milliseconds（秒换算为毫秒）_11/2  "Constant（常量）"
  Constant（常量）_15/1 -> Every20ms（20毫秒更新许可）_16/2  "Constant（常量）"
  Milliseconds（秒换算为毫秒）_11/1 -> RoundTime（按原规则取整）_12/1  "Milliseconds（秒换算为毫秒）"
  RoundTime（按原规则取整）_12/1 -> Phase20（20毫秒相位）_14/1  "RoundTime（按原规则取整）"
  Constant（常量）_13/1 -> Phase20（20毫秒相位）_14/2  "Constant（常量）"
  Phase20（20毫秒相位）_14/1 -> Every20ms（20毫秒更新许可）_16/1  "Phase20（20毫秒相位）"

== system turbo_controller/BoardInput_输入换算与协议解析/In05_Speed（转速来源选择与滤波）/Select（优先级与保持选择）_65 ==
  note: 按优先级决定这一周期输出哪种转速
      |
      | 输入包含20 ms许可、四个来源条件、捕获分母有效标志，两种候选转速，以及上次Speed和等待次数。
      | 处理顺序很重要。
      |
      | 先看20 ms许可：本毫秒不到更新时间，就保持上次Speed和等待次数。
      | 到更新时间后，如果UseMotor成立，直接采用电机反馈Motor，同时等待次数清零。
      | 如果不再使用Motor，但Waiting仍成立，则保持旧Speed，并将等待次数加1，最多等待10次节拍。
      |
      | 等待结束后，先看捕获是否Timeout：超时就输出0。未超时时，Enough和Valid同时成立才采用Capture
      | d；数量不够或分母无效时仍保持Held。
      |
      | 例如电机刚停止给定，不会立刻切到可能还未准备好的捕获值，而先保持约0.2 s。Speed和WaitCount
      | 输出在父级被保存，下一次再作为历史输入，所以不能删除这两条记忆反馈。
  Control（二十毫秒许可）_40 : Inport  OutDataTypeStr=boolean
  UseMotor（电机反馈优先）_41 : Inport  Port=2  OutDataTypeStr=boolean
  Waiting（切换等待中）_42 : Inport  Port=3  OutDataTypeStr=boolean
  Timeout（脉冲已超时）_43 : Inport  Port=4  OutDataTypeStr=boolean
  Enough（间隔数足够）_44 : Inport  Port=5  OutDataTypeStr=boolean
  Valid（估算分母有效）_45 : Inport  Port=6  OutDataTypeStr=boolean
  Motor（电机反馈转速）_46 : Inport  Port=7  OutDataTypeStr=single
  Captured（捕获估算转速）_47 : Inport  Port=8  OutDataTypeStr=single
  Held（上次控制转速）_48 : Inport  Port=9  OutDataTypeStr=single
  WaitCount（上次等待次数）_49 : Inport  Port=10  OutDataTypeStr=uint8
  Add（加减运算）_59 : Sum  SaturateOnIntegerOverflow=on  OutDataTypeStr=Inherit: Same as first input
  AdvanceWait（等待最多十次）_60 : Switch  Criteria=u2 ~= 0  SaturateOnIntegerOverflow=off  InputSameDT=off
  CanEstimate（捕获数据可用）_50 : Logic  IconShape=distinctive  AllPortsSameDT=off  OutDataTypeStr=boolean
  CaptureOrHold（估算有效才更新）_52 : Switch  Criteria=u2 ~= 0  SaturateOnIntegerOverflow=off  InputSameDT=off
  Constant（常量）_51 : Constant  Value=0  OutDataTypeStr=single
  Constant（常量）_57 : Constant  Value=0  OutDataTypeStr=uint8
  Constant（常量）_58 : Constant  OutDataTypeStr=uint8
  MotorResetsWait（电机运行时等待清零）_61 : Switch  Criteria=u2 ~= 0  SaturateOnIntegerOverflow=off  InputSameDT=off
  Priority（优先使用电机反馈）_55 : Switch  Criteria=u2 ~= 0  SaturateOnIntegerOverflow=off  InputSameDT=off
  PulseResult（超时输出零）_53 : Switch  Criteria=u2 ~= 0  SaturateOnIntegerOverflow=off  InputSameDT=off
  Update20ms（其余毫秒保持）_56 : Switch  Criteria=u2 ~= 0  SaturateOnIntegerOverflow=off  InputSameDT=off
  Wait20ms（每二十毫秒更新等待次数）_62 : Switch  Criteria=u2 ~= 0  SaturateOnIntegerOverflow=off  InputSameDT=off
  WaitOrCapture（等待后改用捕获）_54 : Switch  Criteria=u2 ~= 0  SaturateOnIntegerOverflow=off  InputSameDT=off
  Speed（本次控制转速）_63 : Outport
  WaitCount（下次等待次数）_64 : Outport  Port=2
  wires:
  Control（二十毫秒许可）_40/1 -> Update20ms（其余毫秒保持）_56/2, Wait20ms（每二十毫秒更新等待次数）_62/2  "Control（二十毫秒许可）"
  Held（上次控制转速）_48/1 -> Update20ms（其余毫秒保持）_56/3, WaitOrCapture（等待后改用捕获）_54/1, CaptureOrHold（估算有效才更新）_52/3  "Held（上次控制转速）"
  Enough（间隔数足够）_44/1 -> CanEstimate（捕获数据可用）_50/1  "Enough（间隔数足够）"
  UseMotor（电机反馈优先）_41/1 -> MotorResetsWait（电机运行时等待清零）_61/2, Priority（优先使用电机反馈）_55/2  "UseMotor（电机反馈优先）"
  WaitCount（上次等待次数）_49/1 -> Add（加减运算）_59/1, Wait20ms（每二十毫秒更新等待次数）_62/3, AdvanceWait（等待最多十次）_60/3  "WaitCount（上次等待次数）"
  Constant（常量）_58/1 -> Add（加减运算）_59/2  "Constant（常量）"
  Valid（估算分母有效）_45/1 -> CanEstimate（捕获数据可用）_50/2  "Valid（估算分母有效）"
  Constant（常量）_51/1 -> PulseResult（超时输出零）_53/1  "Constant（常量）"
  Update20ms（其余毫秒保持）_56/1 -> Speed（本次控制转速）_63/1  "Update20ms（其余毫秒保持）"
  Captured（捕获估算转速）_47/1 -> CaptureOrHold（估算有效才更新）_52/1  "Captured（捕获估算转速）"
  CanEstimate（捕获数据可用）_50/1 -> CaptureOrHold（估算有效才更新）_52/2  "CanEstimate（捕获数据可用）"
  Timeout（脉冲已超时）_43/1 -> PulseResult（超时输出零）_53/2  "Timeout（脉冲已超时）"
  CaptureOrHold（估算有效才更新）_52/1 -> PulseResult（超时输出零）_53/3  "CaptureOrHold（估算有效才更新）"
  Add（加减运算）_59/1 -> AdvanceWait（等待最多十次）_60/1  "Add（加减运算）"
  Waiting（切换等待中）_42/1 -> AdvanceWait（等待最多十次）_60/2, WaitOrCapture（等待后改用捕获）_54/2  "Waiting（切换等待中）"
  PulseResult（超时输出零）_53/1 -> WaitOrCapture（等待后改用捕获）_54/3  "PulseResult（超时输出零）"
  Constant（常量）_57/1 -> MotorResetsWait（电机运行时等待清零）_61/1  "Constant（常量）"
  AdvanceWait（等待最多十次）_60/1 -> MotorResetsWait（电机运行时等待清零）_61/3  "AdvanceWait（等待最多十次）"
  Motor（电机反馈转速）_46/1 -> Priority（优先使用电机反馈）_55/1  "Motor（电机反馈转速）"
  WaitOrCapture（等待后改用捕获）_54/1 -> Priority（优先使用电机反馈）_55/3  "WaitOrCapture（等待后改用捕获）"
  MotorResetsWait（电机运行时等待清零）_61/1 -> Wait20ms（每二十毫秒更新等待次数）_62/1  "MotorResetsWait（电机运行时等待清零）"
  Priority（优先使用电机反馈）_55/1 -> Update20ms（其余毫秒保持）_56/1  "Priority（优先使用电机反馈）"
  Wait20ms（每二十毫秒更新等待次数）_62/1 -> WaitCount（下次等待次数）_64/1  "Wait20ms（每二十毫秒更新等待次数）"

== system turbo_controller/BoardInput_输入换算与协议解析/In05_Speed（转速来源选择与滤波）/Status（来源与超时判定）_39 ==
  note: 转速来源现在是否可用
      |
      | 这里不计算转速，而把输入整理成四个供Select使用的布尔条件。
      |
      | UseMotor：上一周期电机给定大于0，表示电机仍在被驱动，优先采用电机串口反馈。
      | Waiting：等待次数小于10，表示从电机反馈退出后还在过渡期。等待次数由外层按20 ms节拍推进，10
      | 次约0.2 s。
      | Timeout：当前秒数减最近有效脉冲时间大于0.1 s，表示捕获结果已经不够新鲜。
      | Enough：有效间隔数至少3，保证去掉最大和最小之后还有数据。
      |
      | 例如已有10项间隔，但最后一次脉冲是0.3 s前，Enough虽为真，Timeout也为真，仍不能把旧估速当作
      | 当前转速。四个条件各表达一件事，由后面的Select按优先级合成决定。
  PreviousMotor（上一电机给定）_20 : Inport  OutDataTypeStr=uint16
  Count（有效间隔数）_21 : Inport  Port=2  OutDataTypeStr=uint8
  LastTime（最近脉冲秒数）_22 : Inport  Port=3  OutDataTypeStr=single
  Seconds（当前秒数）_23 : Inport  Port=4  OutDataTypeStr=double
  WaitCount（切换等待次数）_24 : Inport  Port=5  OutDataTypeStr=uint8
  Cast（数据类型转换）_31 : DataTypeConversion  OutDataTypeStr=single  RndMeth=Round
  Constant（常量）_25 : Constant  Value=0  OutDataTypeStr=uint16
  Constant（常量）_28 : Constant  Value=10  OutDataTypeStr=uint8
  Constant（常量）_33 : Constant  Value=single(0.1)  OutDataTypeStr=single
  Constant（常量）_36 : Constant  Value=3  OutDataTypeStr=uint8
  Elapsed（距最近脉冲的秒数）_32 : Sum  Inputs=+-  SaturateOnIntegerOverflow=on  OutDataTypeStr=Inherit: Same as first input
  Enough（至少三个间隔）_37 : RelationalOperator  OutDataTypeStr=boolean  RndMeth=Simplest  InputSameDT=off
  MotorActive（电机给定非零）_26 : RelationalOperator  Operator=>  OutDataTypeStr=boolean  RndMeth=Simplest  InputSameDT=off
  Timeout（超过零点一秒无脉冲）_34 : RelationalOperator  Operator=>  OutDataTypeStr=boolean  RndMeth=Simplest  InputSameDT=off
  WaitTen（等待十次二十毫秒）_29 : RelationalOperator  Operator=<  OutDataTypeStr=boolean  RndMeth=Simplest  InputSameDT=off
  UseMotor（电机反馈优先）_27 : Outport
  Waiting（切换等待尚未完成）_30 : Outport  Port=2
  Timeout（捕获脉冲超时）_35 : Outport  Port=3
  Enough（有效间隔至少三个）_38 : Outport  Port=4
  wires:
  Seconds（当前秒数）_23/1 -> Cast（数据类型转换）_31/1  "Seconds（当前秒数）"
  Count（有效间隔数）_21/1 -> Enough（至少三个间隔）_37/1  "Count（有效间隔数）"
  WaitCount（切换等待次数）_24/1 -> WaitTen（等待十次二十毫秒）_29/1  "WaitCount（切换等待次数）"
  PreviousMotor（上一电机给定）_20/1 -> MotorActive（电机给定非零）_26/1  "PreviousMotor（上一电机给定）"
  Constant（常量）_28/1 -> WaitTen（等待十次二十毫秒）_29/2  "Constant（常量）"
  MotorActive（电机给定非零）_26/1 -> UseMotor（电机反馈优先）_27/1  "MotorActive（电机给定非零）"
  Timeout（超过零点一秒无脉冲）_34/1 -> Timeout（捕获脉冲超时）_35/1  "Timeout（超过零点一秒无脉冲）"
  Constant（常量）_36/1 -> Enough（至少三个间隔）_37/2  "Constant（常量）"
  Constant（常量）_25/1 -> MotorActive（电机给定非零）_26/2  "Constant（常量）"
  Elapsed（距最近脉冲的秒数）_32/1 -> Timeout（超过零点一秒无脉冲）_34/1  "Elapsed（距最近脉冲的秒数）"
  WaitTen（等待十次二十毫秒）_29/1 -> Waiting（切换等待尚未完成）_30/1  "WaitTen（等待十次二十毫秒）"
  Cast（数据类型转换）_31/1 -> Elapsed（距最近脉冲的秒数）_32/1  "Cast（数据类型转换）"
  Enough（至少三个间隔）_37/1 -> Enough（有效间隔至少三个）_38/1  "Enough（至少三个间隔）"
  LastTime（最近脉冲秒数）_22/1 -> Elapsed（距最近脉冲的秒数）_32/2  "LastTime（最近脉冲秒数）"
  Constant（常量）_33/1 -> Timeout（超过零点一秒无脉冲）_34/2  "Constant（常量）"

== system turbo_controller/BoardInput_输入换算与协议解析/In06_Analog（模拟量换算）/TotalTemperature（总温电阻与编码换算）_112 ==
  note: 两路电压怎样反算总温
      |
      | 本模块位于In06_Analog内部，输入仍是完整八项ADC数组，但只用第5和第7项。第5项是测量电路的参
      | 考计数，第7项是温度传感器计数。计算的思路是先恢复电压，再由电路关系求电阻，最后由电阻标定
      | 得到温度。
      |
      | 1 按现有电路比例恢复电压：
      | 参考电压 Vref = 第5项 × 3/4096 × 6/3.3；
      | 传感器电压 Vs = 第7项 × 3/4096；
      | 电压差 ΔV = Vref - Vs，以上单位均为V。
      | 这里的6/3.3是参考支路采用的比例，不能省略。
      |
      | 2 当ΔV大于0.1 V时，采用有效电阻：
      | R = 1000 × Vs / ΔV。
      | 1000来自当前电路换算系数。例子：Vs为1 V、ΔV为1 V时，计算电阻为1000。
      |
      | 3 将电阻换成温度：
      | 原始温度 = 0.25506 × R - 254.987696，单位℃；
      | 输出T0编码 = 原始温度 + 80。
      | 所以输出不是直接摄氏温度。后面ISM/Calibrating_T0会减80，并限制在-70～175 ℃。
      |
      | 4 若ΔV不大于0.1 V，模型不采用这次除法结果，而输出替代电阻9999；分母选择支路也提供安全值，
      | 避免无效路径除零。该替代值继续换算后，会在下一级被限到175 ℃。这条处理没有另外输出“断线告
      | 警”，不能把175 ℃误认为一定是实测温度。
      |
      | 本模块结果经In06_Analog和ControlRate16送入ISM。之后总温用于记录、回传及HuanSuanN温度修正转
      | 速；它没有直接接入Dynamic_Cal的参考温度输入。
  ADC（八路原始采样）_84 : Inport  OutDataTypeStr=uint16
  Add（加减运算）_108 : Sum  Inputs=+-  SaturateOnIntegerOverflow=on  OutDataTypeStr=Inherit: Same as first input
  Cast（数据类型转换）_86 : DataTypeConversion  OutDataTypeStr=single  RndMeth=Round
  Cast（数据类型转换）_92 : DataTypeConversion  OutDataTypeStr=single  RndMeth=Round
  Constant（常量）_100 : Constant  OutDataTypeStr=single
  Constant（常量）_103 : Constant  Value=9999  OutDataTypeStr=single
  Constant（常量）_105 : Constant  Value=single(0.25506)  OutDataTypeStr=single
  Constant（常量）_107 : Constant  Value=single(254.987696)  OutDataTypeStr=single
  Constant（常量）_109 : Constant  Value=80  OutDataTypeStr=single
  Constant（常量）_87 : Constant  Value=3/4096  OutDataTypeStr=single
  Constant（常量）_89 : Constant  Value=single(6/3.3)  OutDataTypeStr=single
  Constant（常量）_93 : Constant  Value=3/4096  OutDataTypeStr=single
  Constant（常量）_96 : Constant  Value=single(0.1)  OutDataTypeStr=single
  Constant（常量）_98 : Constant  Value=1000  OutDataTypeStr=single
  Difference（参考与传感器电压差）_95 : Sum  Inputs=+-  SaturateOnIntegerOverflow=on  OutDataTypeStr=Inherit: Same as first input
  Divide（相除）_102 : Product  Inputs=*/  SaturateOnIntegerOverflow=on  OutDataTypeStr=Inherit: Same as first input
  Multiply（相乘）_106 : Product  Inputs=**  SaturateOnIntegerOverflow=on  OutDataTypeStr=Inherit: Same as first input
  Multiply（相乘）_88 : Product  Inputs=**  SaturateOnIntegerOverflow=on  OutDataTypeStr=Inherit: Same as first input
  Multiply（相乘）_99 : Product  Inputs=**  SaturateOnIntegerOverflow=on  OutDataTypeStr=Inherit: Same as first input
  ReferenceVoltage（总温参考电压）_90 : Product  Inputs=**  SaturateOnIntegerOverflow=on  OutDataTypeStr=Inherit: Same as first input
  Reference（第五路参考计数）_85 : Selector  InputPortWidth=8  IndexOptions=Index vector (dialog)  Indices=5  OutputSizes=1
  Resistance（计算电阻或保留原无效值）_104 : Switch  Criteria=u2 ~= 0  SaturateOnIntegerOverflow=off  InputSameDT=off
  Select（按条件选择）_101 : Switch  Criteria=u2 ~= 0  SaturateOnIntegerOverflow=off  InputSameDT=off
  SensorVoltage（传感器电压）_94 : Product  Inputs=**  SaturateOnIntegerOverflow=on  OutDataTypeStr=Inherit: Same as first input
  Sensor（第七路传感器计数）_91 : Selector  InputPortWidth=8  IndexOptions=Index vector (dialog)  Indices=7  OutputSizes=1
  T0（保留原总温编码公式）_110 : Sum  SaturateOnIntegerOverflow=on  OutDataTypeStr=Inherit: Same as first input
  Valid（电压差大于零点一伏）_97 : RelationalOperator  Operator=>  OutDataTypeStr=boolean  RndMeth=Simplest  InputSameDT=off
  T0（总温编码）_111 : Outport
  wires:
  T0（保留原总温编码公式）_110/1 -> T0（总温编码）_111/1  "T0（保留原总温编码公式）"
  Constant（常量）_109/1 -> T0（保留原总温编码公式）_110/2  "Constant（常量）"
  Add（加减运算）_108/1 -> T0（保留原总温编码公式）_110/1  "Add（加减运算）"
  Constant（常量）_107/1 -> Add（加减运算）_108/2  "Constant（常量）"
  Multiply（相乘）_106/1 -> Add（加减运算）_108/1  "Multiply（相乘）"
  Resistance（计算电阻或保留原无效值）_104/1 -> Multiply（相乘）_106/2  "Resistance（计算电阻或保留原无效值）"
  Constant（常量）_105/1 -> Multiply（相乘）_106/1  "Constant（常量）"
  Constant（常量）_103/1 -> Resistance（计算电阻或保留原无效值）_104/3  "Constant（常量）"
  Divide（相除）_102/1 -> Resistance（计算电阻或保留原无效值）_104/1  "Divide（相除）"
  Select（按条件选择）_101/1 -> Divide（相除）_102/2  "Select（按条件选择）"
  Multiply（相乘）_99/1 -> Divide（相除）_102/1  "Multiply（相乘）"
  Constant（常量）_100/1 -> Select（按条件选择）_101/3  "Constant（常量）"
  Valid（电压差大于零点一伏）_97/1 -> Resistance（计算电阻或保留原无效值）_104/2, Select（按条件选择）_101/2  "Valid（电压差大于零点一伏）"
  Constant（常量）_98/1 -> Multiply（相乘）_99/2  "Constant（常量）"
  Constant（常量）_96/1 -> Valid（电压差大于零点一伏）_97/2  "Constant（常量）"
  Difference（参考与传感器电压差）_95/1 -> Select（按条件选择）_101/1, Valid（电压差大于零点一伏）_97/1  "Difference（参考与传感器电压差）"
  SensorVoltage（传感器电压）_94/1 -> Difference（参考与传感器电压差）_95/2, Multiply（相乘）_99/1  "SensorVoltage（传感器电压）"
  ReferenceVoltage（总温参考电压）_90/1 -> Difference（参考与传感器电压差）_95/1  "ReferenceVoltage（总温参考电压）"
  Constant（常量）_93/1 -> SensorVoltage（传感器电压）_94/2  "Constant（常量）"
  Cast（数据类型转换）_92/1 -> SensorVoltage（传感器电压）_94/1  "Cast（数据类型转换）"
  Sensor（第七路传感器计数）_91/1 -> Cast（数据类型转换）_92/1  "Sensor（第七路传感器计数）"
  Constant（常量）_89/1 -> ReferenceVoltage（总温参考电压）_90/2  "Constant（常量）"
  Multiply（相乘）_88/1 -> ReferenceVoltage（总温参考电压）_90/1  "Multiply（相乘）"
  Constant（常量）_87/1 -> Multiply（相乘）_88/2  "Constant（常量）"
  Cast（数据类型转换）_86/1 -> Multiply（相乘）_88/1  "Cast（数据类型转换）"
  Reference（第五路参考计数）_85/1 -> Cast（数据类型转换）_86/1  "Reference（第五路参考计数）"
  ADC（八路原始采样）_84/1 -> Reference（第五路参考计数）_85/1, Sensor（第七路传感器计数）_91/1  "ADC（八路原始采样）"

== system turbo_controller/BoardOutput_串口封装与阀门时序/Out01_Pump（泵反馈解析与滤波）/Receive（逐字节组帧与保持有效结果）_680 ==
  note: 实际油泵反馈接收流程：按1→2→3→4阅读
      |
      | 第一步只遍历本批有效字节，最多处理64项；第二步识别AA55、收齐22字节，并保存尚未收完的半帧；
      | 第三步确认本字节刚收齐且CRC通过；第四步换算数值并保存最近有效结果。
      |
      | Loop在一次调用内逐字节重复这些步骤，不是每一步各等1 ms。接收数组的Index每批重新遍历，收帧P
      | osition可以跨批保留，两者不是同一个位置。
      |
      | 有效帧第6、7字节合成泵反馈，按0.875旧值+0.125新值更新；没有新帧时不重复滤波。
      |
      | 本次将原有处理块按职责封装，保留原协议、初始化、数据类型、校验和循环行为。各步骤内部可看输
      | 入、公式和例子。
  Rx（本次接收字节）_557 : Inport  OutDataTypeStr=uint8
  Count（本次有效字节数）_558 : Inport  Port=2  OutDataTypeStr=uint32
  Loop（逐项处理循环）_559 : ForIterator  IterationLimit=64  ExternalIncrement=on  IterationVariableDataType=uint32
  Step01_取字节与循环控制 : Subsystem  Description=|
      | 第一步：只处理本批收到的字节
      | 
      | 接收数组最多64项，Count是这次新收到的数量，Loop给出从1开始的Index。Byte=Rx(Index)，Active=(Index≤Count)。
      | 
      | 处理到Index≥Count或Index=64，就把下一循环序号设65，使Loop退出；否则下一序号=Index+1。Count=3只处理第1～3项；Count=0时仍走一次无效项保持路径，但不会把数组旧值加入帧。
      | 
      | 输出Byte和Active给组帧步骤，下一序号反馈Loop。这里不识别帧头，不作CRC，不把Index当作跨批收帧位置。
  Step02_拼帧并保存半帧 : Subsystem  Description=|
      | 第二步：跨多次接收保存半帧
      | 
      | 将本项字节、有效标志、上次候选缓存和上次收帧Position交给Collect。Collect识别AA55并逐项填满22字节，具体规则已在其内部再拆成五步。
      | 
      | 更新后的缓存和Position经原数据类型转换，送回两条记忆块；所以第一次只收到一半，下一批还能接着填，不必从头找AA。输出候选帧与“本字节刚收齐”，交第三步校验。
      | 
      | 候选缓存不等于已接受结果。即使旧缓存里已经有完整内容，没有本次收齐事件也不能再次接受它。这里的记忆按原循环节奏推进，没有增加一个额外的采样周期等待。
  Step03_收齐且校验通过才接受 : Subsystem  Description=|
      | 第三步：刚收齐且CRC通过，才接受新帧
      | 
      | Complete表示这一项字节刚把22字节补齐，先按原类型传给Verify触发校验。Verify对第6～20字节计算CRC16，分别与第21、22字节的高、低校验字节比较。
      | 
      | 最后Accepted=Complete AND Verify通过。这样未收齐的数据不会被采用，Verify上一帧保留的通过状态也不会在没有新Complete时重新接收旧帧。
      | 
      | CRC初值、表和覆盖范围保留原设置。校验失败只让本次Accepted为假；后面的保持步骤继续输出上一有效反馈。本处不作反馈比例换算，不直接生成驱动命令。
  Step04_换算反馈并保持有效结果 : Subsystem  Description=|
      | 第四步：还原泵反馈，只在新有效帧时平滑一次
      | 
      | 第6、7字节高位在前，合成原始反馈=高字节×256+低字节。再计算候选滤波值=0.875×旧输出+0.125×原始反馈。
      | 
      | Accepted为真时才采用候选值并更新Pump记忆，否则保持旧值。例如旧输出800、新有效反馈1000，本次结果825；若接着几个调用没有新有效帧，仍是825，不会反复用旧数据再滤波。
      | 
      | 这里是接收反馈，不是油泵目标设定。输出随后用于上位机回传；串口控制命令仍由独立输出路径生成。
  Speed（当前有效反馈）_679 : Outport
  wires:
  Step04_换算反馈并保持有效结果/1(输出1_最近有效反馈) -> Speed（当前有效反馈）_679/1
  Step01_取字节与循环控制/3(输出3_下一循环序号) -> Loop（逐项处理循环）_559/1
  Step03_收齐且校验通过才接受/1(输出1_本字节接受有效帧) -> Step04_换算反馈并保持有效结果/2(输入2_本字节接受有效帧)  "本字节接受有效帧"
  Step02_拼帧并保存半帧/2(输出2_候选帧缓存) -> Step03_收齐且校验通过才接受/2(输入2_候选帧缓存), Step04_换算反馈并保持有效结果/1(输入1_候选帧缓存)  "候选帧缓存"
  Step02_拼帧并保存半帧/1(输出1_本字节刚收齐) -> Step03_收齐且校验通过才接受/1(输入1_本字节刚收齐)  "本字节刚收齐"
  Step01_取字节与循环控制/2(输出2_本项字节有效) -> Step02_拼帧并保存半帧/2(输入2_本项字节有效)  "本项字节有效"
  Step01_取字节与循环控制/1(输出1_本项字节) -> Step02_拼帧并保存半帧/1(输入1_本项字节)  "本项字节"
  Rx（本次接收字节）_557/1 -> Step01_取字节与循环控制/3(输入3_本批接收数组)  "本批接收数组"
  Count（本次有效字节数）_558/1 -> Step01_取字节与循环控制/2(输入2_本批有效字节数)  "本批有效字节数"
  Loop（逐项处理循环）_559/1 -> Step01_取字节与循环控制/1(输入1_本批循环序号)  "本批循环序号"

== system turbo_controller/BoardOutput_串口封装与阀门时序/Out02_Timing（阀门与点火时序）/AuxValve（副阀周期与开度）_747 ==
  note: 副阀怎样按周期形成开启区间
      |
      | 本模块收到使能Enable、周期计数Cycle、开启计数Open，以及父级给出的偶数毫秒节拍Even。它输出
      | 的是逻辑开启状态On，父级随后才按低有效电路把它取反成引脚电平。
      |
      | 先检查Enable是否非零、Cycle是否非零，两者都成立才允许运行。对Cycle为零的情况，SafeCycle提
      | 供1作为取余用的安全分母，但运行许可仍为假，所以不会因为避免除零而误开阀。
      |
      | 内部Phase记住周期位置，在2 ms节拍内按先归一化、后推进的分支更新。位置到周期末尾通过取余回
      | 到起点；位置小于Open时On为真，其余区间为假。
      |
      | 例如Cycle=30、Open=15，约每60 ms重复一次，其中约30 ms开启；Open=0则没有开启区间，Open不小
      | 于周期时允许区间覆盖整个周期。这里的15是15个2 ms计数，不是15 ms。
      |
      | 禁止使能时按关闭支路处理，不能仅看历史Phase猜测当前输出。位置跨1 ms调用保存，是周期波形成
      | 立所必需的状态。
  Enable（阀门使能）_720 : Inport
  Cycle（周期计数）_721 : Inport  Port=2
  Open（开启计数）_723 : Inport  Port=3
  Even（本毫秒为偶数节拍）_725 : Inport  Port=4  OutDataTypeStr=boolean
  Add（加减运算）_744 : Sum  SaturateOnIntegerOverflow=on  OutDataTypeStr=Inherit: Same as first input
  Advance（奇数毫秒推进一次计数）_745 : Switch  Criteria=u2 ~= 0  SaturateOnIntegerOverflow=off  InputSameDT=off
  Cast（数据类型转换）_722 : DataTypeConversion  OutDataTypeStr=uint32  RndMeth=Round
  Cast（数据类型转换）_724 : DataTypeConversion  OutDataTypeStr=uint32  RndMeth=Round
  Cast（数据类型转换）_734 : DataTypeConversion  OutDataTypeStr=double  RndMeth=Round
  Cast（数据类型转换）_735 : DataTypeConversion  OutDataTypeStr=double  RndMeth=Round
  Cast（数据类型转换）_737 : DataTypeConversion  OutDataTypeStr=uint32  RndMeth=Floor
  Constant（常量）_727 : Constant  Value=0  OutDataTypeStr=uint8
  Constant（常量）_729 : Constant  Value=0  OutDataTypeStr=uint32
  Constant（常量）_732 : Constant  OutDataTypeStr=uint32
  Constant（常量）_738 : Constant  Value=0  OutDataTypeStr=uint32
  Constant（常量）_743 : Constant  OutDataTypeStr=uint32
  CycleValid（周期不为零）_730 : RelationalOperator  Operator=~=  OutDataTypeStr=boolean  RndMeth=Simplest  InputSameDT=off
  Enabled（使能不为零）_728 : RelationalOperator  Operator=~=  OutDataTypeStr=boolean  RndMeth=Simplest  InputSameDT=off
  InsideOpen（当前位于开启区间）_741 : RelationalOperator  Operator=<  OutDataTypeStr=boolean  RndMeth=Simplest  InputSameDT=off
  Phase（跨毫秒保存的周期位置）_726 : UnitDelay  InitialCondition=uint32(0)  SampleTime=-1  HasFrameUpgradeWarning=on
  Running（允许周期运行）_731 : Logic  IconShape=distinctive  AllPortsSameDT=off  OutDataTypeStr=boolean
  SafeCycle（零周期时避免取余异常）_733 : Switch  Criteria=u2 ~= 0  SaturateOnIntegerOverflow=off  InputSameDT=off
  Select（按条件选择）_739 : Switch  Criteria=u2 ~= 0  SaturateOnIntegerOverflow=off  InputSameDT=off
  Store_uint32（按三十二位无符号数保存状态）_537208 : DataTypeConversion  Description=为反馈回路显式指定原程序的状态类型，保持原状态更新节拍。  OutDataTypeStr=uint32  RndMeth=Round
  Update2ms（每两毫秒归一化周期位置）_740 : Switch  Criteria=u2 ~= 0  SaturateOnIntegerOverflow=off  InputSameDT=off
  ValveOn（本毫秒阀门开启）_742 : Logic  IconShape=distinctive  AllPortsSameDT=off  OutDataTypeStr=boolean
  WrapCycle（按周期长度回卷）_736 : Math  Operator=mod
  On（逻辑开启状态）_746 : Outport
  wires:
  ValveOn（本毫秒阀门开启）_742/1 -> On（逻辑开启状态）_746/1  "ValveOn（本毫秒阀门开启）"
  Add（加减运算）_744/1 -> Advance（奇数毫秒推进一次计数）_745/3  "Add（加减运算）"
  Constant（常量）_743/1 -> Add（加减运算）_744/2  "Constant（常量）"
  InsideOpen（当前位于开启区间）_741/1 -> ValveOn（本毫秒阀门开启）_742/2  "InsideOpen（当前位于开启区间）"
  Cast（数据类型转换）_724/1 -> InsideOpen（当前位于开启区间）_741/2  "Cast（数据类型转换）"
  Update2ms（每两毫秒归一化周期位置）_740/1 -> Add（加减运算）_744/1, Advance（奇数毫秒推进一次计数）_745/1, InsideOpen（当前位于开启区间）_741/1  "Update2ms（每两毫秒归一化周期位置）"
  Even（本毫秒为偶数节拍）_725/1 -> Advance（奇数毫秒推进一次计数）_745/2, Update2ms（每两毫秒归一化周期位置）_740/2  "Even（本毫秒为偶数节拍）"
  Select（按条件选择）_739/1 -> Update2ms（每两毫秒归一化周期位置）_740/1  "Select（按条件选择）"
  Constant（常量）_738/1 -> Select（按条件选择）_739/3  "Constant（常量）"
  Running（允许周期运行）_731/1 -> Select（按条件选择）_739/2, ValveOn（本毫秒阀门开启）_742/1  "Running（允许周期运行）"
  Cast（数据类型转换）_737/1 -> Select（按条件选择）_739/1  "Cast（数据类型转换）"
  WrapCycle（按周期长度回卷）_736/1 -> Cast（数据类型转换）_737/1  "WrapCycle（按周期长度回卷）"
  Cast（数据类型转换）_735/1 -> WrapCycle（按周期长度回卷）_736/2  "Cast（数据类型转换）"
  Cast（数据类型转换）_734/1 -> WrapCycle（按周期长度回卷）_736/1  "Cast（数据类型转换）"
  SafeCycle（零周期时避免取余异常）_733/1 -> Cast（数据类型转换）_735/1  "SafeCycle（零周期时避免取余异常）"
  Constant（常量）_732/1 -> SafeCycle（零周期时避免取余异常）_733/3  "Constant（常量）"
  CycleValid（周期不为零）_730/1 -> Running（允许周期运行）_731/2, SafeCycle（零周期时避免取余异常）_733/2  "CycleValid（周期不为零）"
  Enabled（使能不为零）_728/1 -> Running（允许周期运行）_731/1  "Enabled（使能不为零）"
  Constant（常量）_729/1 -> CycleValid（周期不为零）_730/2  "Constant（常量）"
  Cast（数据类型转换）_722/1 -> CycleValid（周期不为零）_730/1, SafeCycle（零周期时避免取余异常）_733/1  "Cast（数据类型转换）"
  Constant（常量）_727/1 -> Enabled（使能不为零）_728/2  "Constant（常量）"
  Enable（阀门使能）_720/1 -> Enabled（使能不为零）_728/1  "Enable（阀门使能）"
  Open（开启计数）_723/1 -> Cast（数据类型转换）_724/1  "Open（开启计数）"
  Cycle（周期计数）_721/1 -> Cast（数据类型转换）_722/1  "Cycle（周期计数）"
  Store_uint32（按三十二位无符号数保存状态）_537208/1 -> Phase（跨毫秒保存的周期位置）_726/1
  Phase（跨毫秒保存的周期位置）_726/1 -> Cast（数据类型转换）_734/1, Update2ms（每两毫秒归一化周期位置）_740/3  "Phase（跨毫秒保存的周期位置）"
  Advance（奇数毫秒推进一次计数）_745/1 -> Store_uint32（按三十二位无符号数保存状态）_537208/1  "Advance（奇数毫秒推进一次计数）"

== system turbo_controller/BoardOutput_串口封装与阀门时序/Out02_Timing（阀门与点火时序）/Ignition（点火九毫秒开一毫秒关）_764 ==
  note: 点火请求怎样形成九开一关的节奏
      |
      | 输入Request是点火请求，非零表示允许点火；它不是已经产生的脉冲。内部Phase按每1 ms调用推进，
      | 在0～9之间循环：
      | 下一位置 = mod(当前位置 + 1,10)。
      |
      | 当请求有效且当前位置小于9时，On=true；位置等于9时On=false。因此每10 ms中前9 ms接通、最后1
      | ms断开，周期约100 Hz，逻辑占空比90%。
      |
      | 请求无效时，输出关闭并把位置清零。下一次请求到来从新周期起点开始，不继续沿用停火前的位置。
      | 输出On交父级FireLow取反，生成低有效点火引脚电平。所以本图“开启”为真与实际引脚为低是同一
      | 动作的两种表示。
      |
      | uint8用于保存0～9的相位；这里先取余再存储，不依赖整数溢出制造周期。
  Request（点火请求）_748 : Inport
  Add（加减运算）_757 : Sum  SaturateOnIntegerOverflow=on  OutDataTypeStr=Inherit: Same as first input
  Cast（数据类型转换）_755 : DataTypeConversion  OutDataTypeStr=double  RndMeth=Round
  Cast（数据类型转换）_760 : DataTypeConversion  OutDataTypeStr=uint8  RndMeth=Floor
  Constant（常量）_750 : Constant  Value=0  OutDataTypeStr=uint8
  Constant（常量）_752 : Constant  Value=9  OutDataTypeStr=uint8
  Constant（常量）_756 : Constant  OutDataTypeStr=double
  Constant（常量）_758 : Constant  Value=10  OutDataTypeStr=double
  Constant（常量）_761 : Constant  Value=0  OutDataTypeStr=uint8
  Enabled（点火请求有效）_751 : RelationalOperator  Operator=~=  OutDataTypeStr=boolean  RndMeth=Simplest  InputSameDT=off
  Ignite（九开一关的点火状态）_754 : Logic  IconShape=distinctive  AllPortsSameDT=off  OutDataTypeStr=boolean
  OnNine（前九毫秒接通）_753 : RelationalOperator  Operator=<  OutDataTypeStr=boolean  RndMeth=Simplest  InputSameDT=off
  Phase（十毫秒点火位置）_749 : UnitDelay  InitialCondition=uint8(0)  SampleTime=-1  HasFrameUpgradeWarning=on
  Stop（无点火请求时位置清零）_762 : Switch  Criteria=u2 ~= 0  SaturateOnIntegerOverflow=off  InputSameDT=off
  Store_uint8（按八位无符号数保存状态）_537230 : DataTypeConversion  Description=为反馈回路显式指定原程序的状态类型，保持原状态更新节拍。  OutDataTypeStr=uint8  RndMeth=Round
  Wrap10（十毫秒循环）_759 : Math  Operator=mod
  On（本毫秒点火接通）_763 : Outport
  wires:
  Constant（常量）_761/1 -> Stop（无点火请求时位置清零）_762/3  "Constant（常量）"
  Constant（常量）_750/1 -> Enabled（点火请求有效）_751/2  "Constant（常量）"
  Request（点火请求）_748/1 -> Enabled（点火请求有效）_751/1  "Request（点火请求）"
  Store_uint8（按八位无符号数保存状态）_537230/1 -> Phase（十毫秒点火位置）_749/1
  Phase（十毫秒点火位置）_749/1 -> Cast（数据类型转换）_755/1, OnNine（前九毫秒接通）_753/1  "Phase（十毫秒点火位置）"
  Constant（常量）_752/1 -> OnNine（前九毫秒接通）_753/2  "Constant（常量）"
  Enabled（点火请求有效）_751/1 -> Stop（无点火请求时位置清零）_762/2, Ignite（九开一关的点火状态）_754/1  "Enabled（点火请求有效）"
  OnNine（前九毫秒接通）_753/1 -> Ignite（九开一关的点火状态）_754/2  "OnNine（前九毫秒接通）"
  Cast（数据类型转换）_755/1 -> Add（加减运算）_757/1  "Cast（数据类型转换）"
  Constant（常量）_756/1 -> Add（加减运算）_757/2  "Constant（常量）"
  Add（加减运算）_757/1 -> Wrap10（十毫秒循环）_759/1  "Add（加减运算）"
  Constant（常量）_758/1 -> Wrap10（十毫秒循环）_759/2  "Constant（常量）"
  Wrap10（十毫秒循环）_759/1 -> Cast（数据类型转换）_760/1  "Wrap10（十毫秒循环）"
  Cast（数据类型转换）_760/1 -> Stop（无点火请求时位置清零）_762/1  "Cast（数据类型转换）"
  Stop（无点火请求时位置清零）_762/1 -> Store_uint8（按八位无符号数保存状态）_537230/1  "Stop（无点火请求时位置清零）"
  Ignite（九开一关的点火状态）_754/1 -> On（本毫秒点火接通）_763/1  "Ignite（九开一关的点火状态）"
